simulink model "sf_atomic_matrix_fixed"  (R2025b)
settings: Solver=FixedStepDiscrete  StartTime=0.0  StopTime=10.0  FixedStep=1  RelTol=1e-3  EnableMultiTasking=on
libraries: sf_atomic_matrix_library x2
settings Model: Creator=The MathWorks, Inc.  LastModifiedBy=The MathWorks, Inc.
settings SolverCC: AlgebraicLoopSolver=TrustRegion
settings DataIOCC: LimitDataPoints=on  SaveFormat=Array  ReturnWorkspaceOutputs=off
settings OptimizationCC: ReuseModelBlockBuffer=off  ExpressionDepthLimit=2147483647.0  LifeSpan=1  EfficientTunableParamExpr=on
settings DebuggingCC: UnderspecifiedInitializationDetection=Classic  MergeDetectMultiDrivingBlocksExec=none  SolverPrmCheckMsg=warning  FcnCallInpInsideContextMsg=warning  UnconnectedInputMsg=warning  UnconnectedOutputMsg=warning  UnconnectedLineMsg=warning  StateNameClashWarn=warning  PregeneratedLibrarySubsystemCodeDiagnostic=none  SFUnexpectedBacktrackingDiag=warning  SFNoUnconditionalDefaultTransitionDiag=warning  SFExecutionAtInitializationDiag=none  ArithmeticOperatorsInVariantConditions=warning
settings HardwareCC: ProdBitPerPointer=32.0  ProdBitPerSizeT=32.0  ProdBitPerPtrDiffT=32.0  ProdLargestAtomicFloat=None  ProdIntDivRoundTo=Undefined  ProdEndianess=Unspecified  ProdWordSize=32.0  ProdHWDeviceType=32-bit Generic
settings ModelReferenceCC: EnableRefExpFcnMdlSchedulingChecks=on  PropagateSignalLabelsOutOfModel=off
settings SFSimCC: SimUseLocalCustomCode=off  SimParseCustomCode=off  MATLABDynamicMemAlloc=off  CustomCodeUndefinedFunction=UseInterfaceOnly
settings RTWCC: SystemTargetFile=ert.tlc  TemplateMakefile=ert_default_tmf  GenerateReport=on  RTWUseLocalCustomCode=off  IncludeHyperlinkInReport=on  LaunchReport=on  GenerateTraceInfo=on  GenerateTraceReport=on  GenerateTraceReportSl=on  GenerateTraceReportSf=on  GenerateTraceReportEml=on  GPUComputeCapability=3.5  Description=Real-Time Workshop Embedded Coder
settings CodeAppCC: IgnoreCustomStorageClasses=off  CustomSymbolStrType=$N$R$M  StateflowObjectComments=on  InternalIdentifier=Classic
settings ERTTargetCC: InlinedParameterPlacement=Hierarchical  ERTCustomFileTemplate=example_file_process.tlc  ConvertIfToSwitch=off  SuppressUnreachableDefaultCases=off  MultiwordLength=2048.0  GenerateSampleERTMain=on  SupportContinuousTime=on
settings ConfigComp: CovMetricSettings=dw  CovSaveCumulativeToWorkspaceVar=on  CovSaveSingleToWorkspaceVar=on  CovExternalEMLEnable=off

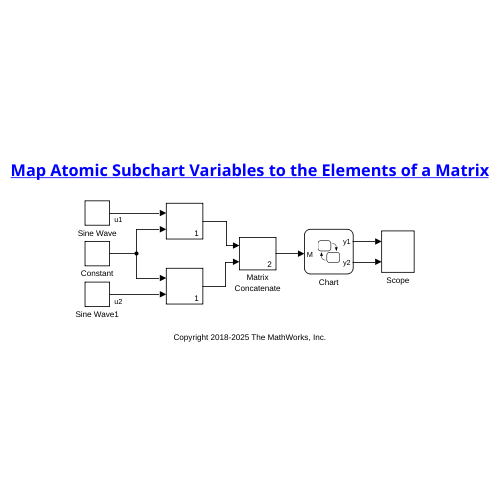
[thumbnail: Simulink's stored preview of the top-level diagram]
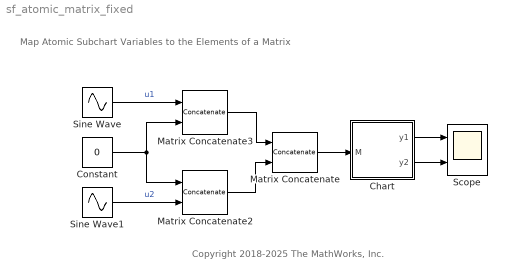
== system sf_atomic_matrix_fixed ==
  note: Copyright 2018-2025 The MathWorks, Inc.
  note: Map Atomic Subchart Variables to the Elements of a Matrix
  Chart : Stateflow chart  TreatAsAtomicUnit=on
  Constant : Constant  Value=0
  Matrix Concatenate : Concatenate  Mode=Multidimensional array  ConcatenateDimension=2
  Matrix Concatenate2 : Concatenate  Mode=Multidimensional array
  Matrix Concatenate3 : Concatenate  Mode=Multidimensional array
  Scope : Scope  NumInputPorts=2
      settings: ActiveDisplayYMinimum=-5  ActiveDisplayYMaximum=5
  Sine Wave : Sin  SampleTime=0
  Sine Wave1 : Sin  Frequency=2  SampleTime=0
  wires:
  Chart/1(y1) -> Scope/1
  Chart/2(y2) -> Scope/2
  Constant/1 -> Matrix Concatenate3/2, Matrix Concatenate2/1
  Sine Wave/1 -> Matrix Concatenate3/1  "u1"
  Sine Wave1/1 -> Matrix Concatenate2/2  "u2"
  Matrix Concatenate3/1 -> Matrix Concatenate/1
  Matrix Concatenate2/1 -> Matrix Concatenate/2
  Matrix Concatenate/1 -> Chart/1(M)

== stateflow chart sf_atomic_matrix_fixed/Chart ==
  state A [parallel]
    settings: executionOrder=1
  state B [parallel]
    settings: executionOrder=2
  data: u1 function_input double; u1 function_input double; y1 output double; y2 output double; M input double size=[2 2]
